simulink model "StampFly_StudentBlocks"  (R2026b)
settings: Solver=VariableStepAuto
undefined symbols (not defined in the file): Bottom, Official
(part 2 of 6)

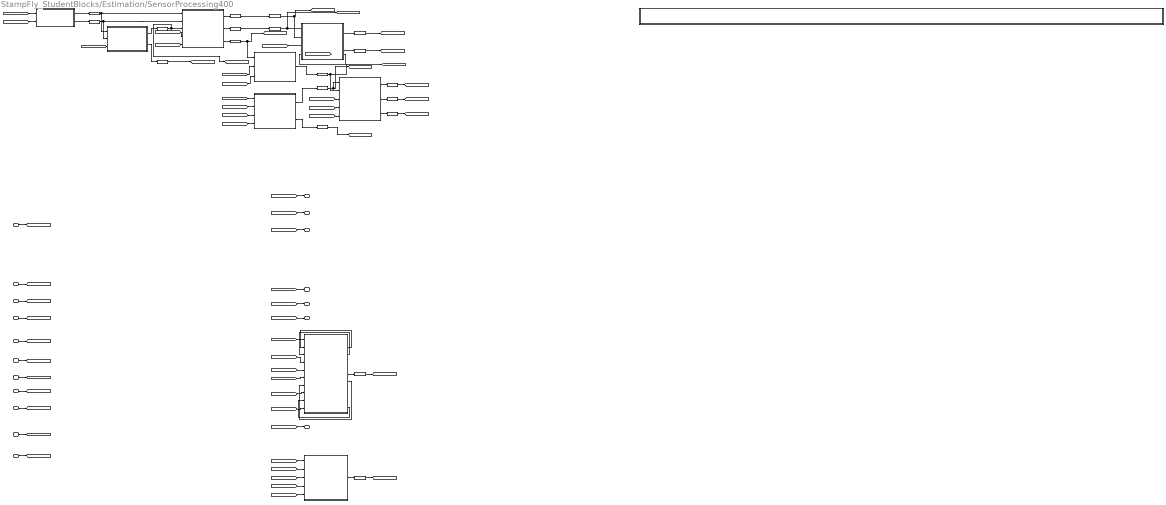
== system StampFly_StudentBlocks/Estimation/SensorProcessing400 ==
  AccelMps2 : Inport
  GyroRps : Inport  Port=2
  ToFmm : Inport  Port=3
  ToFNew : Inport  Port=4
  Voltage : Inport  Port=5
  PreviousMode : Inport  Port=6
  AltFlag : Inport  Port=7
  Dt : Inport  Port=8
  AHRSReset : Inport  Port=9
  ParkingReset : Inport  Port=10
  FlipFlag : Inport  Port=11
  Accel3Size : SignalSpecification  OutDataTypeStr=single  Dimensions=3
  AltitudeKalman : Stateflow chart  Description=高度・鉛直速度・バイアス  TreatAsAtomicUnit=on
      settings: AttributesFormatString=|
      | 高度 Kalman 推定
      | 高度・鉛直速度・バイアス
  Gyro3Size : SignalSpecification  OutDataTypeStr=single  Dimensions=3
  IMUAxisConversion : Stateflow chart  Description=BMI270 → 航空機座標  TreatAsAtomicUnit=on
      settings: AttributesFormatString=|
      | 軸・単位の変換
      | BMI270 → 航空機座標
  IMUBiasCalibration : Stateflow chart  Description=800サンプルでオフセット推定  TreatAsAtomicUnit=on
      settings: AttributesFormatString=|
      | 静止時の校正
      | 800サンプルでオフセット推定
  IMUFiltering : Stateflow chart  Description=校正値を引き一次フィルター  TreatAsAtomicUnit=on
      settings: AttributesFormatString=|
      | IMU フィルター
      | 校正値を引き一次フィルター
  MadgwickAttitude : Stateflow chart  Description=400 Hz / Roll・Pitch・Yaw  TreatAsAtomicUnit=on
      settings: AttributesFormatString=|
      | Madgwick 姿勢推定
      | 400 Hz / Roll・Pitch・Yaw
  ModelExplanation : Subsystem  Description=400 Hz の推定処理：軸変換 → 静止校正 → フィルター → 姿勢推定。下段は ToF と鉛直加速度から高度・上下速度を推定。各ブロックを個別に差し替え可能。
      mask Display: disp('説明\n400 Hz の推定処理：軸変換 → 静止校正 → フィルター → 姿勢推定。下段は ToF と鉛直加速度から高度・上下速度を推定。各ブロックを個別に差し替え可能。')
  SensorDiagnosticPack : Stateflow chart  Description=記録用にまとめる  TreatAsAtomicUnit=on
      settings: AttributesFormatString=|
      | 推定器の診断信号
      | 記録用にまとめる
  SensorFlags : Stateflow chart  Description=距離異常・過加速度・低電圧  TreatAsAtomicUnit=on
      settings: AttributesFormatString=|
      | センサーの状態判定
      | 距離異常・過加速度・低電圧
  ToFHoldOutlierFilter : Stateflow chart  Description=新着距離を判定 / 旧値を保持  TreatAsAtomicUnit=on
      settings: AttributesFormatString=|
      | ToF 保持・外れ値処理
      | 新着距離を判定 / 旧値を保持
  VerticalAcceleration : Stateflow chart  Description=重力成分を除去・フィルター  TreatAsAtomicUnit=on
      settings: AttributesFormatString=|
      | 鉛直加速度
      | 重力成分を除去・フィルター
  spec117_1 : SignalSpecification  OutDataTypeStr=single  Dimensions=3
  spec117_2 : SignalSpecification  OutDataTypeStr=single  Dimensions=3
  spec118_1 : SignalSpecification  OutDataTypeStr=single  Dimensions=4
  spec118_2 : SignalSpecification  OutDataTypeStr=uint16  Dimensions=1
  spec119_1 : SignalSpecification  OutDataTypeStr=single  Dimensions=3
  spec119_2 : SignalSpecification  OutDataTypeStr=single  Dimensions=3
  spec119_3 : SignalSpecification  OutDataTypeStr=single  Dimensions=1
  spec120_1 : SignalSpecification  OutDataTypeStr=single  Dimensions=3
  spec120_2 : SignalSpecification  OutDataTypeStr=single  Dimensions=4
  spec121_1 : SignalSpecification  OutDataTypeStr=single  Dimensions=1
  spec122_1 : SignalSpecification  OutDataTypeStr=single  Dimensions=1
  spec122_2 : SignalSpecification  OutDataTypeStr=int16  Dimensions=1
  spec123_1 : SignalSpecification  OutDataTypeStr=single  Dimensions=1
  spec123_2 : SignalSpecification  OutDataTypeStr=single  Dimensions=1
  spec123_3 : SignalSpecification  OutDataTypeStr=single  Dimensions=1
  spec124_1 : SignalSpecification  OutDataTypeStr=uint8  Dimensions=3
  spec125_1 : SignalSpecification  OutDataTypeStr=single  Dimensions=8
  Attitude3 : Outport  OutDataTypeStr=single  PortDimensions=3
  Rates3 : Outport  Port=2  OutDataTypeStr=single  PortDimensions=3
  Altitude : Outport  Port=3
  Velocity : Outport  Port=4
  Flags3 : Outport  Port=5
  Quaternion4 : Outport  Port=6  OutDataTypeStr=single  PortDimensions=4
  Diagnostics8 : Outport  Port=7
  wires:
  IMUFiltering/2(gf) -> spec119_2/1
  IMUFiltering/1(af) -> spec119_1/1
  IMUBiasCalibration/2(count) -> spec118_2/1
  ToFHoldOutlierFilter/1(alt) -> spec122_1/1
  ToFHoldOutlierFilter/2(raw) -> spec122_2/1
  IMUBiasCalibration/1(offset) -> spec118_1/1
  IMUAxisConversion/2(g) -> spec117_2/1
  IMUAxisConversion/1(a) -> spec117_1/1
  spec117_1/1 -> IMUFiltering/1(a), IMUBiasCalibration/1(a)
  spec117_2/1 -> IMUBiasCalibration/2(g), IMUFiltering/2(g)
  SensorDiagnosticPack/1(diag) -> spec125_1/1
  SensorFlags/1(flags) -> spec124_1/1
  spec125_1/1 -> [diag_S125P1]
  spec124_1/1 -> [flags_S124P1]
  AHRSReset/1 -> [AHRSReset_S83P1]
  FlipFlag/1 -> [FlipFlag_S561P1]
  AltFlag/1 -> [AltFlag_S81P1]
  Voltage/1 -> [Voltage_S79P1]
  ParkingReset/1 -> [ParkingReset_S84P1]
  Dt/1 -> [Dt_S82P1]
  PreviousMode/1 -> [PreviousMode_S80P1]
  ToFNew/1 -> [ToFNew_S78P1]
  ToFmm/1 -> [ToFmm_S77P1]
  GyroRps/1 -> [GyroRps_S76P1]
  AccelMps2/1 -> [AccelMps2_S75P1]
  [Voltage_S79P1] -> SensorFlags/3(voltage)
  [PreviousMode_S80P1] -> SensorFlags/4(mode)
  [AltFlag_S81P1] -> SensorFlags/5(altFlag)
  [Dt_S82P1] -> SensorFlags/8(dt)
  [ParkingReset_S84P1] -> SensorFlags/9(parkingReset)
  [FlipFlag_S561P1] -> SensorFlags/10(flipFlag)
  [af_S119P1] -> SensorFlags/1(accel)
  [gf_S119P2] -> Rates3/1
  [offset_S118P1] -> SensorDiagnosticPack/4(offset)
  [count_S118P2] -> SensorDiagnosticPack/5(count)
  [azd_S119P3] -> SensorFlags/2(azd)
  [a_S120P1] -> Attitude3/1
  [q_S120P2] -> Quaternion4/1
  [az_S121P1] -> SensorDiagnosticPack/1(az)
  [alt_S122P1] -> SensorDiagnosticPack/3(alt)
  [raw_S122P2] -> SensorFlags/7(rawRange)
  [height_S123P1] -> SensorFlags/6(height)
  [height_S123P1] -> Altitude/1
  [velocity_S123P2] -> Velocity/1
  [bias_S123P3] -> SensorDiagnosticPack/2(bias)
  [flags_S124P1] -> Flags3/1
  [diag_S125P1] -> Diagnostics8/1
  spec122_2/1 -> [raw_S122P2]
  spec120_1/1 -> [a_S120P1]
  spec118_2/1 -> [count_S118P2]
  spec118_1/1 -> IMUFiltering/3(offset), [offset_S118P1]
  [AccelMps2_S75P1] -> IMUAxisConversion/1(accelMps2)
  [GyroRps_S76P1] -> IMUAxisConversion/2(gyroRps)
  [ToFmm_S77P1] -> ToFHoldOutlierFilter/1(mm)
  [ToFNew_S78P1] -> ToFHoldOutlierFilter/2(fresh)
  [PreviousMode_S80P1] -> IMUFiltering/4(mode)
  [PreviousMode_S80P1] -> IMUBiasCalibration/3(mode)
  [PreviousMode_S80P1] -> ToFHoldOutlierFilter/3(mode)
  [Dt_S82P1] -> ToFHoldOutlierFilter/4(dt)
  [Dt_S82P1] -> IMUFiltering/5(dt)
  [AHRSReset_S83P1] -> MadgwickAttitude/4(reset)
  [PreviousMode_S80P1] -> MadgwickAttitude/3(mode)
  spec120_2/1 -> [q_S120P2]
  MadgwickAttitude/1(a) -> spec120_1/1
  MadgwickAttitude/2(q) -> spec120_2/1
  VerticalAcceleration/1(az) -> spec121_1/1
  IMUFiltering/3(azd) -> spec119_3/1
  spec119_1/1 -> Accel3Size/1
  spec119_2/1 -> Gyro3Size/1
  spec121_1/1 -> [az_S121P1], AltitudeKalman/2(az)
  spec119_3/1 -> [azd_S119P3], VerticalAcceleration/1(azd)
  Accel3Size/1 -> MadgwickAttitude/2(accel), [af_S119P1]
  Gyro3Size/1 -> MadgwickAttitude/1(rates), [gf_S119P2]
  [PreviousMode_S80P1] -> VerticalAcceleration/2(mode)
  [Dt_S82P1] -> VerticalAcceleration/3(dt)
  [ParkingReset_S84P1] -> AltitudeKalman/5(parkingReset)
  [Dt_S82P1] -> AltitudeKalman/4(dt)
  [PreviousMode_S80P1] -> AltitudeKalman/3(mode)
  spec122_1/1 -> [alt_S122P1], AltitudeKalman/1(alt)
  spec123_1/1 -> [height_S123P1]
  spec123_2/1 -> [velocity_S123P2]
  spec123_3/1 -> [bias_S123P3]
  AltitudeKalman/1(height) -> spec123_1/1
  AltitudeKalman/2(velocity) -> spec123_2/1
  AltitudeKalman/3(bias) -> spec123_3/1

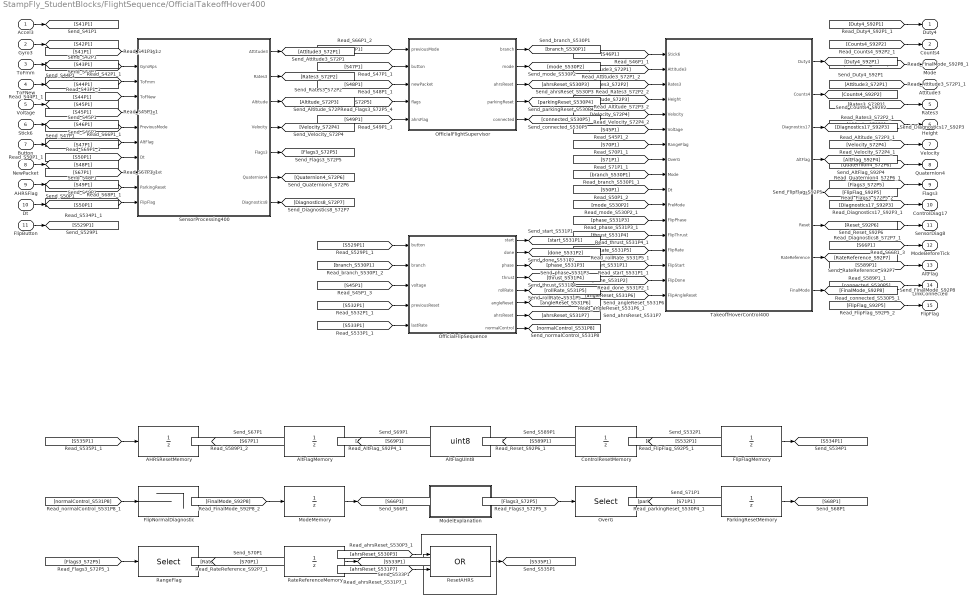
== system StampFly_StudentBlocks/FlightSequence/OfficialTakeoffHover400 ==
  Accel3 : Inport
  Gyro3 : Inport  Port=2
  ToFmm : Inport  Port=3
  ToFNew : Inport  Port=4
  Voltage : Inport  Port=5
  Stick6 : Inport  Port=6
  Button : Inport  Port=7
  NewPacket : Inport  Description=新しいJoyStickパケットをこの周期で受信したか。通信中のフラグとは異なります。  Port=8
  AHRSFlag : Inport  Port=9
  Dt : Inport  Port=10
  FlipButton : Inport  Port=11
  AHRSResetMemory : UnitDelay  InitialCondition=false  SampleTime=Official.Step
  AltFlagMemory : UnitDelay  InitialCondition=uint8(0)  SampleTime=Official.Step
  AltFlagUInt8 : DataTypeConversion  OutDataTypeStr=uint8  SaturateOnIntegerOverflow=off  RndMeth=Floor
  ControlResetMemory : UnitDelay  InitialCondition=false  SampleTime=Official.Step
  FlipFlagMemory : UnitDelay  InitialCondition=uint8(0)  SampleTime=Official.Step
  FlipNormalDiagnostic : Terminator
  ModeMemory : UnitDelay  InitialCondition=uint8(0)  SampleTime=Official.Step
  ModelExplanation : Subsystem  Description=センサー入力 → 推定 → 状態管理 → PID → モーター指令。各ブロックを個別に編集できます。
      mask Display: disp('説明\nセンサー入力 → 推定 → 状態管理 → PID → モーター指令。各ブロックを個別に編集できます。')
  OfficialFlightSupervisor : Stateflow chart  TreatAsAtomicUnit=on
  OfficialFlipSequence : Stateflow chart  TreatAsAtomicUnit=on
  OverG : Selector  InputPortWidth=3  IndexOptions=Index vector (dialog)  Indices=1  OutputSizes=1
  ParkingResetMemory : UnitDelay  InitialCondition=false  SampleTime=Official.Step
  RangeFlag : Selector  InputPortWidth=3  IndexOptions=Index vector (dialog)  Indices=2  OutputSizes=1
  RateReferenceMemory : UnitDelay  InitialCondition=zeros(3,1,'single')  SampleTime=Official.Step
  ResetAHRS : Logic  Operator=OR  AllPortsSameDT=off  OutDataTypeStr=boolean
  SensorProcessing400 : Subsystem  Description=センサー処理：軸変換、800点校正、フィルター、Madgwick、ToF保持/外れ値、高度Kalman、状態フラグを機能別に配置します。
      mask Display: disp('SensorProcessing400\nダブルクリックで内部を編集')
  TakeoffHoverControl400 : Subsystem  Description=飛行制御：目標値→誤差→高度PID/速度PID/姿勢PID/角速度PID→推力制限→ミキサー→8bit化。PIDの内部は標準演算ブロックです。
      mask Display: disp('TakeoffHoverControl400\nダブルクリックで内部を編集')
  Duty4 : Outport
  Counts4 : Outport  Port=2
  Mode : Outport  Port=3
  Attitude3 : Outport  Port=4
  Rates3 : Outport  Port=5
  Height : Outport  Port=6
  Velocity : Outport  Port=7
  Quaternion4 : Outport  Port=8
  Flags3 : Outport  Port=9
  ControlDiag17 : Outport  Port=10
  SensorDiag8 : Outport  Port=11
  ModeBeforeTick : Outport  Port=12
  AltFlag : Outport  Port=13
  LinkConnected : Outport  Port=14
  FlipFlag : Outport  Port=15
  wires:
  TakeoffHoverControl400/8(FinalMode) -> [FinalMode_S92P8]
  TakeoffHoverControl400/7(RateReference) -> [RateReference_S92P7]
  TakeoffHoverControl400/6(Reset) -> [Reset_S92P6]
  TakeoffHoverControl400/5(FlipFlag) -> [FlipFlag_S92P5]
  TakeoffHoverControl400/3(Diagnostics17) -> [Diagnostics17_S92P3]
  TakeoffHoverControl400/2(Counts4) -> [Counts4_S92P2]
  TakeoffHoverControl400/1(Duty4) -> [Duty4_S92P1]
  AltFlagUInt8/1 -> [S589P1]
  ModeMemory/1 -> [S66P1]
  AltFlagMemory/1 -> [S69P1]
  AHRSResetMemory/1 -> [S67P1]
  ParkingResetMemory/1 -> [S68P1]
  SensorProcessing400/5(Flags3) -> [Flags3_S72P5]
  SensorProcessing400/3(Altitude) -> [Altitude_S72P3]
  SensorProcessing400/1(Attitude3) -> [Attitude3_S72P1]
  SensorProcessing400/2(Rates3) -> [Rates3_S72P2]
  SensorProcessing400/4(Velocity) -> [Velocity_S72P4]
  RangeFlag/1 -> [S70P1]
  OverG/1 -> [S71P1]
  SensorProcessing400/6(Quaternion4) -> [Quaternion4_S72P6]
  SensorProcessing400/7(Diagnostics8) -> [Diagnostics8_S72P7]
  ControlResetMemory/1 -> [S532P1]
  RateReferenceMemory/1 -> [S533P1]
  OfficialFlipSequence/3(phase) -> [phase_S531P3]
  OfficialFlipSequence/4(thrust) -> [thrust_S531P4]
  OfficialFlipSequence/5(rollRate) -> [rollRate_S531P5]
  OfficialFlipSequence/1(start) -> [start_S531P1]
  OfficialFlipSequence/2(done) -> [done_S531P2]
  OfficialFlipSequence/6(angleReset) -> [angleReset_S531P6]
  TakeoffHoverControl400/4(AltFlag) -> [AltFlag_S92P4]
  FlipFlagMemory/1 -> [S534P1]
  OfficialFlipSequence/7(ahrsReset) -> [ahrsReset_S531P7]
  ResetAHRS/1 -> [S535P1]
  OfficialFlipSequence/8(normalControl) -> [normalControl_S531P8]
  [S41P1] -> SensorProcessing400/1(AccelMps2)
  [S42P1] -> SensorProcessing400/2(GyroRps)
  [S43P1] -> SensorProcessing400/3(ToFmm)
  [S44P1] -> SensorProcessing400/4(ToFNew)
  [S45P1] -> SensorProcessing400/5(Voltage)
  [S45P1] -> TakeoffHoverControl400/6(Voltage)
  [S45P1] -> OfficialFlipSequence/3(voltage)
  [S46P1] -> TakeoffHoverControl400/1(Stick6)
  [S50P1] -> SensorProcessing400/8(Dt)
  [S50P1] -> TakeoffHoverControl400/10(Dt)
  [S529P1] -> OfficialFlipSequence/1(button)
  [S67P1] -> SensorProcessing400/9(AHRSReset)
  [S69P1] -> SensorProcessing400/7(AltFlag)
  [S589P1] -> AltFlag/1
  [S589P1] -> AltFlagMemory/1
  [S532P1] -> OfficialFlipSequence/4(previousReset)
  [S534P1] -> SensorProcessing400/11(FlipFlag)
  [S66P1] -> SensorProcessing400/6(PreviousMode)
  [S66P1] -> ModeBeforeTick/1
  [branch_S530P1] -> TakeoffHoverControl400/9(Mode)
  [branch_S530P1] -> OfficialFlipSequence/2(branch)
  [mode_S530P2] -> TakeoffHoverControl400/11(PreMode)
  [ahrsReset_S530P3] -> ResetAHRS/1
  [parkingReset_S530P4] -> ParkingResetMemory/1
  [connected_S530P5] -> LinkConnected/1
  [start_S531P1] -> TakeoffHoverControl400/15(FlipStart)
  [done_S531P2] -> TakeoffHoverControl400/16(FlipDone)
  [phase_S531P3] -> TakeoffHoverControl400/12(FlipPhase)
  [thrust_S531P4] -> TakeoffHoverControl400/13(FlipThrust)
  [rollRate_S531P5] -> TakeoffHoverControl400/14(FlipRate)
  [angleReset_S531P6] -> TakeoffHoverControl400/17(FlipAngleReset)
  [ahrsReset_S531P7] -> ResetAHRS/2
  [normalControl_S531P8] -> FlipNormalDiagnostic/1
  [S71P1] -> TakeoffHoverControl400/8(OverG)
  [S68P1] -> SensorProcessing400/10(ParkingReset)
  [S70P1] -> TakeoffHoverControl400/7(RangeFlag)
  [S533P1] -> OfficialFlipSequence/5(lastRate)
  [S535P1] -> AHRSResetMemory/1
  [Attitude3_S72P1] -> Attitude3/1
  [Attitude3_S72P1] -> TakeoffHoverControl400/2(Attitude3)
  [Rates3_S72P2] -> Rates3/1
  [Rates3_S72P2] -> TakeoffHoverControl400/3(Rates3)
  [Altitude_S72P3] -> Height/1
  [Altitude_S72P3] -> TakeoffHoverControl400/4(Height)
  [Velocity_S72P4] -> Velocity/1
  [Velocity_S72P4] -> TakeoffHoverControl400/5(Velocity)
  [Flags3_S72P5] -> RangeFlag/1
  [Flags3_S72P5] -> Flags3/1
  [Flags3_S72P5] -> OverG/1
  [Quaternion4_S72P6] -> Quaternion4/1
  [Diagnostics8_S72P7] -> SensorDiag8/1
  [Duty4_S92P1] -> Duty4/1
  [Counts4_S92P2] -> Counts4/1
  [Diagnostics17_S92P3] -> ControlDiag17/1
  [AltFlag_S92P4] -> AltFlagUInt8/1
  [FlipFlag_S92P5] -> FlipFlagMemory/1
  [FlipFlag_S92P5] -> FlipFlag/1
  [Reset_S92P6] -> ControlResetMemory/1
  [RateReference_S92P7] -> RateReferenceMemory/1
  [FinalMode_S92P8] -> Mode/1
  [FinalMode_S92P8] -> ModeMemory/1
  [Flags3_S72P5] -> OfficialFlightSupervisor/4(flags)
  [S66P1] -> OfficialFlightSupervisor/1(previousMode)
  [S49P1] -> OfficialFlightSupervisor/5(ahrsFlag)
  [S48P1] -> OfficialFlightSupervisor/3(newPacket)
  [S47P1] -> OfficialFlightSupervisor/2(button)
  OfficialFlightSupervisor/3(ahrsReset) -> [ahrsReset_S530P3]
  OfficialFlightSupervisor/5(connected) -> [connected_S530P5]
  OfficialFlightSupervisor/4(parkingReset) -> [parkingReset_S530P4]
  OfficialFlightSupervisor/2(mode) -> [mode_S530P2]
  OfficialFlightSupervisor/1(branch) -> [branch_S530P1]
  Stick6/1 -> [S46P1]
  Accel3/1 -> [S41P1]
  Gyro3/1 -> [S42P1]
  ToFmm/1 -> [S43P1]
  ToFNew/1 -> [S44P1]
  Voltage/1 -> [S45P1]
  Dt/1 -> [S50P1]
  Button/1 -> [S47P1]
  NewPacket/1 -> [S48P1]
  AHRSFlag/1 -> [S49P1]
  FlipButton/1 -> [S529P1]

== system StampFly_StudentBlocks/LoggingAndStatus/DataLogger50 ==
  Accel3 : Inport
  Gyro3 : Inport  Port=2
  IMUFresh : Inport  Port=3
  TimeSec : Inport  Port=4
  BottomMm : Inport  Port=5
  ToFNew : Inport  Port=6
  ToFStatus : Inport  Port=7
  BatteryV : Inport  Port=8
  BatteryValid : Inport  Port=9
  Duty4 : Inport  Port=10
  Mode : Inport  Port=11
  Attitude3 : Inport  Port=12
  Height : Inport  Port=13
  Velocity : Inport  Port=14
  ControlDiag17 : Inport  Port=15
  SensorDiag8 : Inport  Port=16
  ToFInfo4 : Inport  Port=17
  CopiedLoggerSFI8_50 : MATLABSystem  Description=50 Hz SFI8記録：下向きToF距離[m]と状態、ToFValid=(距離>0かつ状態0)。ToFFreshは前回の記録から測定完了数が変化したかで判定。無効時も数値ペイロードと状態を保存し、UIは無効データをNaNで表示。Optical FlowはNaN/無効を保存。高度はSimulinkのKalman出力。  Priority=200  System=official.LoggerPacker50  SimulateUsing=Code generation
      mask Type: official.LoggerPacker50
  ESPNowLogger50 : MATLABSystem  Description=ESP-NOWログ：コピーした受信機のログ形式を使います。送信キュー成功と相手の受信成功は別です。  Priority=221  System=imu.ESPNowIMUTx  Channel=uint8( 3 )  SimulateUsing=Code generation
      mask Type: imu.ESPNowIMUTx
  ModelExplanation : Subsystem  Description=50 Hz SFI8記録：下向きToF距離[m]と状態、ToFValid=(距離>0かつ状態0)。ToFFreshは前回の記録から測定完了数が変化したかで判定。無効時も数値ペイロードと状態を保存し、UIは無効データをNaNで表示。Optical FlowはNaN/無効を保存。高度はSimulinkのKalman出力。
      mask Display: disp('説明\n50 Hz SFI8記録：下向きToF距離[m]と状態、ToFValid=(距離>0かつ状態0)。ToFFreshは前回の記録から測定完了数が変化したかで判定。無効時も数値ペイロードと状態を保存し、UIは無効データをNaNで表示。Optical FlowはNaN/無効を保存。高度はSimulinkのKalman出力。')
  QueuedUSBLogger50 : MATLABSystem  Description=USB送信：待ち時間0でキューへ投入し、別タスクから送信。PCのMATロガーで保存します。  Priority=220  System=official.USBLogger50  SimulateUsing=Code generation
      mask Type: official.USBLogger50
  USBDrops : Outport
  RadioQueued : Outport  Port=2
  LEDMode : Outport  Port=3
  wires:
  Accel3/1 -> CopiedLoggerSFI8_50/1
  Gyro3/1 -> CopiedLoggerSFI8_50/2
  IMUFresh/1 -> CopiedLoggerSFI8_50/3
  TimeSec/1 -> CopiedLoggerSFI8_50/4
  BottomMm/1 -> CopiedLoggerSFI8_50/5
  ToFNew/1 -> CopiedLoggerSFI8_50/6
  ToFStatus/1 -> CopiedLoggerSFI8_50/7
  BatteryV/1 -> CopiedLoggerSFI8_50/8
  BatteryValid/1 -> CopiedLoggerSFI8_50/9
  Duty4/1 -> CopiedLoggerSFI8_50/10
  Mode/1 -> CopiedLoggerSFI8_50/11
  Attitude3/1 -> CopiedLoggerSFI8_50/12
  Height/1 -> CopiedLoggerSFI8_50/13
  Velocity/1 -> CopiedLoggerSFI8_50/14
  ControlDiag17/1 -> CopiedLoggerSFI8_50/15
  SensorDiag8/1 -> CopiedLoggerSFI8_50/16
  ToFInfo4/1 -> CopiedLoggerSFI8_50/17
  CopiedLoggerSFI8_50/1 -> QueuedUSBLogger50/1, ESPNowLogger50/1
  QueuedUSBLogger50/1 -> USBDrops/1
  ESPNowLogger50/1 -> RadioQueued/1
  ESPNowLogger50/2 -> LEDMode/1

== system StampFly_StudentBlocks/LoggingAndStatus/JoyStickTelemetry40 ==
  AltFlag : Inport
  Mode : Inport  Port=2
  FrontMm : Inport  Port=3
  TimeSec : Inport  Port=4
  Dt : Inport  Port=5
  Attitude3 : Inport  Port=6
  Rates3 : Inport  Port=7
  ControlDiag17 : Inport  Port=8
  Accel3 : Inport  Port=9
  BatteryV : Inport  Port=10
  Duty4 : Inport  Port=11
  Height : Inport  Port=12
  SensorDiag8 : Inport  Port=13
  Velocity : Inport  Port=14
  ModelExplanation : Subsystem  Description=JoyStickへ公式テレメトリを40 Hzで返信。高度はSimulinkのKalman出力。前向きToFは無効（0）。
      mask Display: disp('説明\nJoyStickへ公式テレメトリを40 Hzで返信。高度はSimulinkのKalman出力。前向きToFは無効（0）。')
  OfficialHeaderGains20 : Constant  Value=single([.65;.7;.01;.125;.95;.7;.025;.125;3;.8;.01;.125;5;4;.04;.125;5;4;.04;.125])
  OfficialJoyTelemetry40 : MATLABSystem  Description=公式JoyStickへ40 Hzで高度・電圧・姿勢・モード等を返信します。  Priority=240  System=official.RadioTelemetryWrite40  SimulateUsing=Code generation
      mask Type: official.RadioTelemetryWrite40
  OfficialTelemetryValues : Stateflow chart  TreatAsAtomicUnit=on
  Sent : Outport
  wires:
  OfficialJoyTelemetry40/1 -> Sent/1
  Velocity/1 -> OfficialTelemetryValues/11(v)
  SensorDiag8/1 -> OfficialTelemetryValues/10(sd)
  Height/1 -> OfficialTelemetryValues/9(z)
  Duty4/1 -> OfficialTelemetryValues/8(duty)
  BatteryV/1 -> OfficialTelemetryValues/7(voltage)
  Accel3/1 -> OfficialTelemetryValues/6(accel)
  ControlDiag17/1 -> OfficialTelemetryValues/5(cd)
  Rates3/1 -> OfficialTelemetryValues/4(r)
  Attitude3/1 -> OfficialTelemetryValues/3(a)
  Dt/1 -> OfficialTelemetryValues/2(dt)
  TimeSec/1 -> OfficialTelemetryValues/1(t)
  FrontMm/1 -> OfficialJoyTelemetry40/5
  Mode/1 -> OfficialJoyTelemetry40/4
  AltFlag/1 -> OfficialJoyTelemetry40/3
  OfficialHeaderGains20/1 -> OfficialJoyTelemetry40/2
  OfficialTelemetryValues/1(values) -> OfficialJoyTelemetry40/1

== system StampFly_StudentBlocks/LoggingAndStatus/StatusOutputs400 ==
  Stick6 : Inport
  SensorFlags3 : Inport  Port=2
  ModeBeforeTick : Inport  Port=3
  AltFlag : Inport  Port=4
  FlipFlag : Inport  Port=5
  PacketError : Inport  Port=6
  AHRSFlag : Inport  Port=7
  ControlMode : Selector  InputPortWidth=6  IndexOptions=Index vector (dialog)  Indices=5  OutputSizes=1
  LowVoltageCount : Selector  InputPortWidth=3  IndexOptions=Index vector (dialog)  Indices=3  OutputSizes=1
  ModelExplanation : Subsystem  Description=公式のモード・姿勢制御方式・高度制御・Flip・低電圧・通信エラーからLED色とブザー周波数を決定。ハードウェアはキュー送出のみ。
      mask Display: disp('説明\n公式のモード・姿勢制御方式・高度制御・Flip・低電圧・通信エラーからLED色とブザー周波数を決定。ハードウェアはキュー送出のみ。')
  StatusIndicators400 : Stateflow chart  TreatAsAtomicUnit=on
  StatusWrite400 : MATLABSystem  System=official.StatusWrite400  SimulateUsing=Code generation
      mask Type: official.StatusWrite400
  UserButton400 : MATLABSystem  System=official.UserButton400  SimulateUsing=Code generation
      mask Type: official.UserButton400
  wires:
  Stick6/1 -> ControlMode/1
  SensorFlags3/1 -> LowVoltageCount/1
  ModeBeforeTick/1 -> StatusIndicators400/1(mode)
  ControlMode/1 -> StatusIndicators400/2(controlMode)
  AltFlag/1 -> StatusIndicators400/3(altFlag)
  FlipFlag/1 -> StatusIndicators400/4(flipFlag)
  LowVoltageCount/1 -> StatusIndicators400/5(lowVoltage)
  PacketError/1 -> StatusIndicators400/6(rcError)
  AHRSFlag/1 -> StatusIndicators400/7(ahrsFlag)
  UserButton400/1 -> StatusIndicators400/8(button)
  StatusIndicators400/1(color1) -> StatusWrite400/1
  StatusIndicators400/2(color2) -> StatusWrite400/2
  StatusIndicators400/3(tone) -> StatusWrite400/3
  StatusIndicators400/4(restart) -> StatusWrite400/4

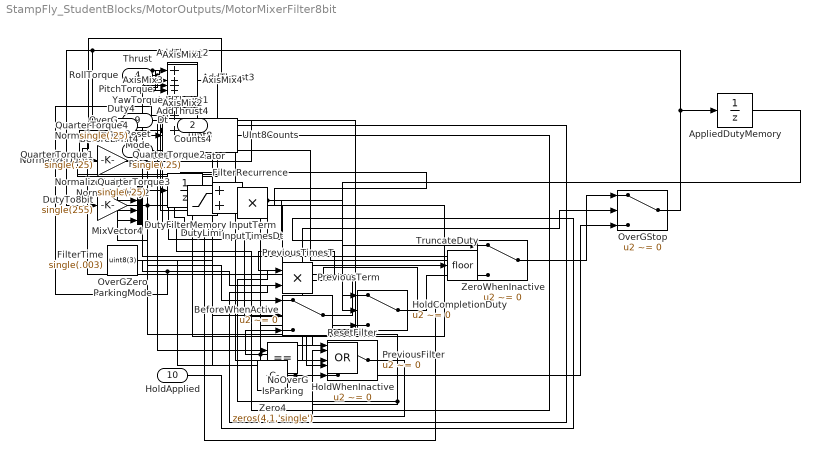
== system StampFly_StudentBlocks/MotorOutputs/MotorMixerFilter8bit ==
  Thrust : Inport
  RollTorque : Inport  Port=2
  PitchTorque : Inport  Port=3
  YawTorque : Inport  Port=4
  Run : Inport  Port=5
  Reset : Inport  Port=6
  OverG : Inport  Port=7
  Mode : Inport  Port=8
  Dt : Inport  Port=9
  HoldApplied : Inport  Port=10
  AddThrust{1..4} (4 alike) : Sum
  AppliedDutyMemory : UnitDelay  InitialCondition=zeros(4,1,'single')  SampleTime=Official.Step
  AxisMix1 : Sum  Inputs=-++
  AxisMix2 : Sum  Inputs=++-
  AxisMix3 : Sum  Inputs=---
  AxisMix4 : Sum  Inputs=+-+
  BeforeWhenActive : Switch  Criteria=u2 ~= 0  SaturateOnIntegerOverflow=off  InputSameDT=off
  DutyFilterMemory : UnitDelay  InitialCondition=zeros(4,1,'single')  SampleTime=Official.Step
  DutyLimit : Saturate  UpperLimit=single(.95)  LowerLimit=single(0)
  DutyTo8bit : Gain  Gain=single(255)
  FilterDenominator : Sum
  FilterRecurrence : Sum
  FilterTime : Constant  Value=single(.003)
  HoldCompletionDuty : Switch  Criteria=u2 ~= 0  SaturateOnIntegerOverflow=off  InputSameDT=off
  HoldWhenInactive : Switch  Criteria=u2 ~= 0  SaturateOnIntegerOverflow=off  InputSameDT=off
  InputTerm : Product  Inputs=*/
  InputTimesDt : Product
  IsParking : RelationalOperator  Operator===  OutDataTypeStr=boolean  RndMeth=Simplest  InputSameDT=off
  MixVector4 : Mux
  NoOverG : RelationalOperator  Operator===  OutDataTypeStr=boolean  RndMeth=Simplest  InputSameDT=off
  NormalizeDuty{1..4} (4 alike) : Gain  Gain=1/3.7  OutDataTypeStr=single
  OverGStop : Switch  Criteria=u2 ~= 0  SaturateOnIntegerOverflow=off  InputSameDT=off
  OverGZero : Constant  Value=uint8(0)
  ParkingMode : Constant  Value=uint8(3)
  PreviousFilter : Switch  Criteria=u2 ~= 0  SaturateOnIntegerOverflow=off  InputSameDT=off
  PreviousTerm : Product  Inputs=*/
  PreviousTimesT : Product
  QuarterTorque{1..4} (4 alike) : Gain  Gain=single(.25)
  ResetFilter : Logic  Operator=OR  AllPortsSameDT=off  OutDataTypeStr=boolean
  TruncateDuty : Rounding
  UInt8Counts : DataTypeConversion  OutDataTypeStr=uint8  SaturateOnIntegerOverflow=off  RndMeth=Floor
  Zero4 : Constant  Value=zeros(4,1,'single')
  ZeroWhenInactive : Switch  Criteria=u2 ~= 0  SaturateOnIntegerOverflow=off  InputSameDT=off
  Duty4 : Outport
  Counts4 : Outport  Port=2
  BeforeLimit4 : Outport  Port=3
  wires:
  RollTorque/1 -> AxisMix2/1, AxisMix3/1, AxisMix1/1, AxisMix4/1
  PitchTorque/1 -> AxisMix1/2, AxisMix2/2, AxisMix3/2, AxisMix4/2
  YawTorque/1 -> AxisMix2/3, AxisMix1/3, AxisMix3/3, AxisMix4/3
  AxisMix1/1 -> QuarterTorque1/1
  Thrust/1 -> AddThrust2/1, AddThrust1/1, AddThrust3/1, AddThrust4/1
  QuarterTorque1/1 -> AddThrust1/2
  AddThrust1/1 -> NormalizeDuty1/1
  AxisMix2/1 -> QuarterTorque2/1
  QuarterTorque2/1 -> AddThrust2/2
  AddThrust2/1 -> NormalizeDuty2/1
  AxisMix3/1 -> QuarterTorque3/1
  QuarterTorque3/1 -> AddThrust3/2
  AddThrust3/1 -> NormalizeDuty3/1
  AxisMix4/1 -> QuarterTorque4/1
  QuarterTorque4/1 -> AddThrust4/2
  AddThrust4/1 -> NormalizeDuty4/1
  Zero4/1 -> OverGStop/3, PreviousFilter/1, BeforeWhenActive/3, HoldCompletionDuty/3
  ResetFilter/1 -> PreviousFilter/2
  DutyFilterMemory/1 -> PreviousFilter/3
  FilterTime/1 -> PreviousTimesT/2, FilterDenominator/1
  PreviousFilter/1 -> PreviousTimesT/1, HoldWhenInactive/3
  PreviousTimesT/1 -> PreviousTerm/1
  FilterDenominator/1 -> PreviousTerm/2, InputTerm/2
  PreviousTerm/1 -> FilterRecurrence/1
  InputTerm/1 -> FilterRecurrence/2
  FilterRecurrence/1 -> DutyLimit/1, HoldWhenInactive/1
  Run/1 -> BeforeWhenActive/2, HoldWhenInactive/2, ZeroWhenInactive/2
  HoldWhenInactive/1 -> DutyFilterMemory/1
  DutyLimit/1 -> ZeroWhenInactive/1
  ZeroWhenInactive/1 -> OverGStop/1
  NoOverG/1 -> OverGStop/2
  OverGStop/1 -> AppliedDutyMemory/1, DutyTo8bit/1, Duty4/1
  DutyTo8bit/1 -> TruncateDuty/1
  TruncateDuty/1 -> UInt8Counts/1
  UInt8Counts/1 -> Counts4/1
  BeforeWhenActive/1 -> BeforeLimit4/1
  NormalizeDuty1/1 -> MixVector4/1
  NormalizeDuty2/1 -> MixVector4/2
  NormalizeDuty3/1 -> MixVector4/3
  NormalizeDuty4/1 -> MixVector4/4
  MixVector4/1 -> InputTimesDt/1, BeforeWhenActive/1
  AppliedDutyMemory/1 -> HoldCompletionDuty/1
  HoldApplied/1 -> HoldCompletionDuty/2
  HoldCompletionDuty/1 -> ZeroWhenInactive/3
  OverGZero/1 -> NoOverG/2
  OverG/1 -> NoOverG/1
  InputTimesDt/1 -> InputTerm/1
  Dt/1 -> FilterDenominator/2, InputTimesDt/2
  Reset/1 -> ResetFilter/2
  IsParking/1 -> ResetFilter/1
  ParkingMode/1 -> IsParking/2
  Mode/1 -> IsParking/1

== system StampFly_StudentBlocks/MotorOutputs/MotorOutputs400 ==
  Counts4 : Inport
  ModelExplanation : Subsystem  Description=入力 Counts4 は FR / FL / RR / RL。LEDCキャリア150 kHz指定・8 bit、指令更新400 Hz。ベンチは定数Enable=falseとAllowMotorOutput=falseで実出力ゼロ。
      mask Display: disp('説明\n入力 Counts4 は FR / FL / RR / RL。LEDCキャリア150 kHz指定・8 bit、指令更新400 Hz。ベンチは定数Enable=falseとAllowMotorOutput=falseで実出力ゼロ。')
  MotorOutputDisabled : Constant  Value=false  SampleTime=Official.Step
  PWM150kHz8bit : MATLABSystem  Description=モーター書き込み：150 kHz指定、8 bit、FR/FL/RR/RL=GPIO42/5/41/10。実機ベンチではAllowMotorOutput=falseかつEnable=false、出力0です。  Priority=100  System=official.MotorPWM400  SampleTime=Official.Step  AllowMotorOutput=false  SimulateUsing=Code generation
      mask Type: official.MotorPWM400
  AppliedCounts4 : Outport
  PWMInfo4 : Outport  Port=2
  wires:
  Counts4/1 -> PWM150kHz8bit/1
  MotorOutputDisabled/1 -> PWM150kHz8bit/2
  PWM150kHz8bit/1 -> AppliedCounts4/1
  PWM150kHz8bit/2 -> PWMInfo4/1

== system StampFly_StudentBlocks/Controllers/TakeoffHoverControl400/AltitudePID ==
  Error : Inport
  Dt : Inport  Port=2
  Enable : Inport  Port=3
  Reset : Inport  Port=4
  PreviousError : Inport  Port=5
  ApplyKp : Product
  DMemory : UnitDelay  InitialCondition=single(0)  SampleTime=Official.Step
  DerivativeDenominator : Sum
  DerivativeErrorProduct : Product
  DerivativeErrorTerm : Product  Inputs=*/
  DerivativePreviousNumerator : Sum  Inputs=+-
  DerivativeUpdate : Sum
  DivideTi : Product  Inputs=*/
  EMemory : UnitDelay  InitialCondition=single(0)  SampleTime=Official.Step
  ErrorDifference : Sum  Inputs=+-
  ErrorPair : Sum
  ErrorPairDt : Product
  Eta : Constant  Value=single(0.125)
  EtaTd : Product
  HalfIntegral : Gain  Gain=single(.5)
  IMemory : UnitDelay  InitialCondition=single(0)  SampleTime=Official.Step
  IntegralLimit : Saturate  UpperLimit=single(30000)  LowerLimit=single(-30000)
  IntegralUpdate : Sum
  Kp : Constant  Value=single(0.379999995)
  PIDTerms : Sum  Inputs=+++
  PreviousDerivativeProduct : Product
  PreviousDerivativeTerm : Product  Inputs=*/
  Select_dnext : Switch  Criteria=u2 ~= 0  SaturateOnIntegerOverflow=off  InputSameDT=off
  Select_dp : Switch  Criteria=u2 ~= 0  SaturateOnIntegerOverflow=off  InputSameDT=off
  Select_enext : Switch  Criteria=u2 ~= 0  SaturateOnIntegerOverflow=off  InputSameDT=off
  Select_ep : Switch  Criteria=u2 ~= 0  SaturateOnIntegerOverflow=off  InputSameDT=off
  Select_inext : Switch  Criteria=u2 ~= 0  SaturateOnIntegerOverflow=off  InputSameDT=off
  Select_ip : Switch  Criteria=u2 ~= 0  SaturateOnIntegerOverflow=off  InputSameDT=off
  Select_output : Switch  Criteria=u2 ~= 0  SaturateOnIntegerOverflow=off  InputSameDT=off
  Select_ynext : Switch  Criteria=u2 ~= 0  SaturateOnIntegerOverflow=off  InputSameDT=off
  Td : Constant  Value=single(0.5)
  Ti : Constant  Value=single(10)
  TwiceEtaTd : Gain  Gain=single(2)
  TwiceTd : Gain  Gain=single(2)
  YMemory : UnitDelay  InitialCondition=single(0)  SampleTime=Official.Step
  Zero : Constant  Value=single(0)
  Output : Outport
  wires:
  Select_output/1 -> Output/1
  Select_ynext/1 -> YMemory/1
  YMemory/1 -> Select_ynext/3, Select_output/3
  ApplyKp/1 -> Select_ynext/1, Select_output/1
  Select_enext/1 -> EMemory/1
  Select_dnext/1 -> DMemory/1
  Select_inext/1 -> IMemory/1
  Enable/1 -> Select_inext/2, Select_dnext/2, Select_enext/2, Select_ynext/2, Select_output/2
  PIDTerms/1 -> ApplyKp/2
  Kp/1 -> ApplyKp/1
  DerivativeUpdate/1 -> PIDTerms/3, Select_dnext/1
  IntegralLimit/1 -> PIDTerms/2, Select_inext/1
  DerivativeErrorTerm/1 -> DerivativeUpdate/2
  PreviousDerivativeTerm/1 -> DerivativeUpdate/1
  DerivativeErrorProduct/1 -> DerivativeErrorTerm/1
  ErrorDifference/1 -> DerivativeErrorProduct/2
  TwiceTd/1 -> DerivativeErrorProduct/1
  DerivativeDenominator/1 -> PreviousDerivativeTerm/2, DerivativeErrorTerm/2
  PreviousDerivativeProduct/1 -> PreviousDerivativeTerm/1
  Select_dp/1 -> PreviousDerivativeProduct/2, Select_dnext/3
  DerivativePreviousNumerator/1 -> PreviousDerivativeProduct/1
  TwiceEtaTd/1 -> DerivativePreviousNumerator/1, DerivativeDenominator/1
  EtaTd/1 -> TwiceEtaTd/1
  Td/1 -> EtaTd/2, TwiceTd/1
  Eta/1 -> EtaTd/1
  IntegralUpdate/1 -> IntegralLimit/1
  DivideTi/1 -> IntegralUpdate/2
  Select_ip/1 -> Select_inext/3, IntegralUpdate/1
  Ti/1 -> DivideTi/2
  HalfIntegral/1 -> DivideTi/1
  ErrorPairDt/1 -> HalfIntegral/1
  ErrorPair/1 -> ErrorPairDt/2
  Dt/1 -> ErrorPairDt/1, DerivativeDenominator/2, DerivativePreviousNumerator/2
  Select_ep/1 -> Select_enext/3, ErrorPair/2, ErrorDifference/2
  Error/1 -> ErrorPair/1, ErrorDifference/1, PIDTerms/1, Select_enext/1
  EMemory/1 -> Select_ep/3
  PreviousError/1 -> Select_ep/1
  DMemory/1 -> Select_dp/3
  IMemory/1 -> Select_ip/3
  Reset/1 -> Select_ip/2, Select_dp/2, Select_ep/2
  Zero/1 -> Select_ip/1, Select_dp/1

== system StampFly_StudentBlocks/Controllers/TakeoffHoverControl400/ModelExplanation ==

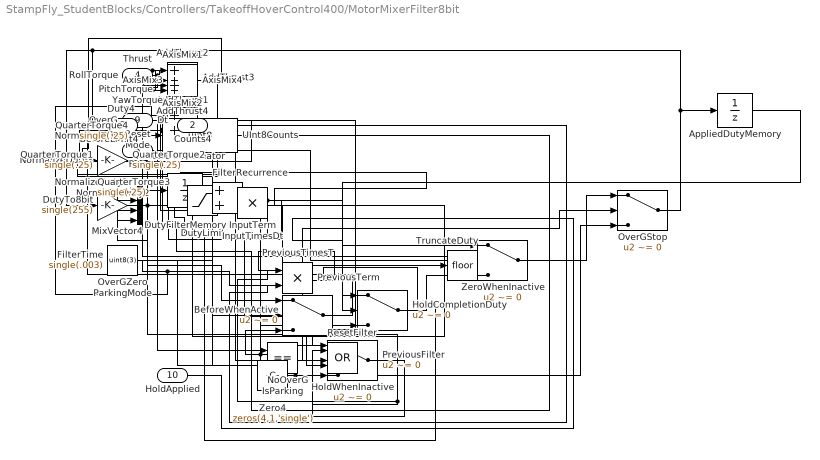
== system StampFly_StudentBlocks/Controllers/TakeoffHoverControl400/MotorMixerFilter8bit ==
  Thrust : Inport
  RollTorque : Inport  Port=2
  PitchTorque : Inport  Port=3
  YawTorque : Inport  Port=4
  Run : Inport  Port=5
  Reset : Inport  Port=6
  OverG : Inport  Port=7
  Mode : Inport  Port=8
  Dt : Inport  Port=9
  HoldApplied : Inport  Port=10
  AddThrust{1..4} (4 alike) : Sum
  AppliedDutyMemory : UnitDelay  InitialCondition=zeros(4,1,'single')  SampleTime=Official.Step
  AxisMix1 : Sum  Inputs=-++
  AxisMix2 : Sum  Inputs=++-
  AxisMix3 : Sum  Inputs=---
  AxisMix4 : Sum  Inputs=+-+
  BeforeWhenActive : Switch  Criteria=u2 ~= 0  SaturateOnIntegerOverflow=off  InputSameDT=off
  DutyFilterMemory : UnitDelay  InitialCondition=zeros(4,1,'single')  SampleTime=Official.Step
  DutyLimit : Saturate  UpperLimit=single(.95)  LowerLimit=single(0)
  DutyTo8bit : Gain  Gain=single(255)
  FilterDenominator : Sum
  FilterRecurrence : Sum
  FilterTime : Constant  Value=single(.003)
  HoldCompletionDuty : Switch  Criteria=u2 ~= 0  SaturateOnIntegerOverflow=off  InputSameDT=off
  HoldWhenInactive : Switch  Criteria=u2 ~= 0  SaturateOnIntegerOverflow=off  InputSameDT=off
  InputTerm : Product  Inputs=*/
  InputTimesDt : Product
  IsParking : RelationalOperator  Operator===  OutDataTypeStr=boolean  RndMeth=Simplest  InputSameDT=off
  MixVector4 : Mux
  NoOverG : RelationalOperator  Operator===  OutDataTypeStr=boolean  RndMeth=Simplest  InputSameDT=off
  NormalizeDuty{1..4} (4 alike) : Gain  Gain=1/3.7  OutDataTypeStr=single
  OverGStop : Switch  Criteria=u2 ~= 0  SaturateOnIntegerOverflow=off  InputSameDT=off
  OverGZero : Constant  Value=uint8(0)
  ParkingMode : Constant  Value=uint8(3)
  PreviousFilter : Switch  Criteria=u2 ~= 0  SaturateOnIntegerOverflow=off  InputSameDT=off
  PreviousTerm : Product  Inputs=*/
  PreviousTimesT : Product
  QuarterTorque{1..4} (4 alike) : Gain  Gain=single(.25)
  ResetFilter : Logic  Operator=OR  AllPortsSameDT=off  OutDataTypeStr=boolean
  TruncateDuty : Rounding
  UInt8Counts : DataTypeConversion  OutDataTypeStr=uint8  SaturateOnIntegerOverflow=off  RndMeth=Floor
  Zero4 : Constant  Value=zeros(4,1,'single')
  ZeroWhenInactive : Switch  Criteria=u2 ~= 0  SaturateOnIntegerOverflow=off  InputSameDT=off
  Duty4 : Outport
  Counts4 : Outport  Port=2
  BeforeLimit4 : Outport  Port=3
  wires:
  RollTorque/1 -> AxisMix2/1, AxisMix3/1, AxisMix1/1, AxisMix4/1
  PitchTorque/1 -> AxisMix1/2, AxisMix2/2, AxisMix3/2, AxisMix4/2
  YawTorque/1 -> AxisMix2/3, AxisMix1/3, AxisMix3/3, AxisMix4/3
  AxisMix1/1 -> QuarterTorque1/1
  Thrust/1 -> AddThrust2/1, AddThrust1/1, AddThrust3/1, AddThrust4/1
  QuarterTorque1/1 -> AddThrust1/2
  AddThrust1/1 -> NormalizeDuty1/1
  AxisMix2/1 -> QuarterTorque2/1
  QuarterTorque2/1 -> AddThrust2/2
  AddThrust2/1 -> NormalizeDuty2/1
  AxisMix3/1 -> QuarterTorque3/1
  QuarterTorque3/1 -> AddThrust3/2
  AddThrust3/1 -> NormalizeDuty3/1
  AxisMix4/1 -> QuarterTorque4/1
  QuarterTorque4/1 -> AddThrust4/2
  AddThrust4/1 -> NormalizeDuty4/1
  Zero4/1 -> OverGStop/3, PreviousFilter/1, BeforeWhenActive/3, HoldCompletionDuty/3
  ResetFilter/1 -> PreviousFilter/2
  DutyFilterMemory/1 -> PreviousFilter/3
  FilterTime/1 -> PreviousTimesT/2, FilterDenominator/1
  PreviousFilter/1 -> PreviousTimesT/1, HoldWhenInactive/3
  PreviousTimesT/1 -> PreviousTerm/1
  FilterDenominator/1 -> PreviousTerm/2, InputTerm/2
  PreviousTerm/1 -> FilterRecurrence/1
  InputTerm/1 -> FilterRecurrence/2
  FilterRecurrence/1 -> DutyLimit/1, HoldWhenInactive/1
  Run/1 -> BeforeWhenActive/2, HoldWhenInactive/2, ZeroWhenInactive/2
  HoldWhenInactive/1 -> DutyFilterMemory/1
  DutyLimit/1 -> ZeroWhenInactive/1
  ZeroWhenInactive/1 -> OverGStop/1
  NoOverG/1 -> OverGStop/2
  OverGStop/1 -> AppliedDutyMemory/1, DutyTo8bit/1, Duty4/1
  DutyTo8bit/1 -> TruncateDuty/1
  TruncateDuty/1 -> UInt8Counts/1
  UInt8Counts/1 -> Counts4/1
  BeforeWhenActive/1 -> BeforeLimit4/1
  NormalizeDuty1/1 -> MixVector4/1
  NormalizeDuty2/1 -> MixVector4/2
  NormalizeDuty3/1 -> MixVector4/3
  NormalizeDuty4/1 -> MixVector4/4
  MixVector4/1 -> InputTimesDt/1, BeforeWhenActive/1
  AppliedDutyMemory/1 -> HoldCompletionDuty/1
  HoldApplied/1 -> HoldCompletionDuty/2
  HoldCompletionDuty/1 -> ZeroWhenInactive/3
  OverGZero/1 -> NoOverG/2
  OverG/1 -> NoOverG/1
  InputTimesDt/1 -> InputTerm/1
  Dt/1 -> FilterDenominator/2, InputTimesDt/2
  Reset/1 -> ResetFilter/2
  IsParking/1 -> ResetFilter/1
  ParkingMode/1 -> IsParking/2
  Mode/1 -> IsParking/1

== system StampFly_StudentBlocks/Controllers/TakeoffHoverControl400/PitchAnglePID ==
  Error : Inport
  Dt : Inport  Port=2
  Enable : Inport  Port=3
  Reset : Inport  Port=4
  PreviousError : Inport  Port=5
  ApplyKp : Product
  DMemory : UnitDelay  InitialCondition=single(0)  SampleTime=Official.Step
  DerivativeDenominator : Sum
  DerivativeErrorProduct : Product
  DerivativeErrorTerm : Product  Inputs=*/
  DerivativePreviousNumerator : Sum  Inputs=+-
  DerivativeUpdate : Sum
  DivideTi : Product  Inputs=*/
  EMemory : UnitDelay  InitialCondition=single(0)  SampleTime=Official.Step
  ErrorDifference : Sum  Inputs=+-
  ErrorPair : Sum
  ErrorPairDt : Product
  Eta : Constant  Value=single(0.125)
  EtaTd : Product
  HalfIntegral : Gain  Gain=single(.5)
  IMemory : UnitDelay  InitialCondition=single(0)  SampleTime=Official.Step
  IntegralLimit : Saturate  UpperLimit=single(30000)  LowerLimit=single(-30000)
  IntegralUpdate : Sum
  Kp : Constant  Value=single(5)
  PIDTerms : Sum  Inputs=+++
  PreviousDerivativeProduct : Product
  PreviousDerivativeTerm : Product  Inputs=*/
  Select_dnext : Switch  Criteria=u2 ~= 0  SaturateOnIntegerOverflow=off  InputSameDT=off
  Select_dp : Switch  Criteria=u2 ~= 0  SaturateOnIntegerOverflow=off  InputSameDT=off
  Select_enext : Switch  Criteria=u2 ~= 0  SaturateOnIntegerOverflow=off  InputSameDT=off
  Select_ep : Switch  Criteria=u2 ~= 0  SaturateOnIntegerOverflow=off  InputSameDT=off
  Select_inext : Switch  Criteria=u2 ~= 0  SaturateOnIntegerOverflow=off  InputSameDT=off
  Select_ip : Switch  Criteria=u2 ~= 0  SaturateOnIntegerOverflow=off  InputSameDT=off
  Select_output : Switch  Criteria=u2 ~= 0  SaturateOnIntegerOverflow=off  InputSameDT=off
  Select_ynext : Switch  Criteria=u2 ~= 0  SaturateOnIntegerOverflow=off  InputSameDT=off
  Td : Constant  Value=single(0.0399999991)
  Ti : Constant  Value=single(4)
  TwiceEtaTd : Gain  Gain=single(2)
  TwiceTd : Gain  Gain=single(2)
  YMemory : UnitDelay  InitialCondition=single(0)  SampleTime=Official.Step
  Zero : Constant  Value=single(0)
  Output : Outport
  wires:
  Enable/1 -> Select_output/2, Select_inext/2, Select_dnext/2, Select_enext/2, Select_ynext/2
  ApplyKp/1 -> Select_ynext/1, Select_output/1
  YMemory/1 -> Select_ynext/3, Select_output/3
  Select_ynext/1 -> YMemory/1
  Select_output/1 -> Output/1
  Select_enext/1 -> EMemory/1
  Select_dnext/1 -> DMemory/1
  Select_inext/1 -> IMemory/1
  PIDTerms/1 -> ApplyKp/2
  Kp/1 -> ApplyKp/1
  DerivativeUpdate/1 -> PIDTerms/3, Select_dnext/1
  IntegralLimit/1 -> PIDTerms/2, Select_inext/1
  DerivativeErrorTerm/1 -> DerivativeUpdate/2
  PreviousDerivativeTerm/1 -> DerivativeUpdate/1
  DerivativeErrorProduct/1 -> DerivativeErrorTerm/1
  ErrorDifference/1 -> DerivativeErrorProduct/2
  TwiceTd/1 -> DerivativeErrorProduct/1
  DerivativeDenominator/1 -> PreviousDerivativeTerm/2, DerivativeErrorTerm/2
  PreviousDerivativeProduct/1 -> PreviousDerivativeTerm/1
  Select_dp/1 -> PreviousDerivativeProduct/2, Select_dnext/3
  DerivativePreviousNumerator/1 -> PreviousDerivativeProduct/1
  TwiceEtaTd/1 -> DerivativePreviousNumerator/1, DerivativeDenominator/1
  EtaTd/1 -> TwiceEtaTd/1
  Td/1 -> EtaTd/2, TwiceTd/1
  Eta/1 -> EtaTd/1
  IntegralUpdate/1 -> IntegralLimit/1
  DivideTi/1 -> IntegralUpdate/2
  Select_ip/1 -> Select_inext/3, IntegralUpdate/1
  Ti/1 -> DivideTi/2
  HalfIntegral/1 -> DivideTi/1
  ErrorPairDt/1 -> HalfIntegral/1
  ErrorPair/1 -> ErrorPairDt/2
  Dt/1 -> ErrorPairDt/1, DerivativeDenominator/2, DerivativePreviousNumerator/2
  Select_ep/1 -> Select_enext/3, ErrorPair/2, ErrorDifference/2
  Error/1 -> ErrorPair/1, ErrorDifference/1, PIDTerms/1, Select_enext/1
  EMemory/1 -> Select_ep/3
  PreviousError/1 -> Select_ep/1
  DMemory/1 -> Select_dp/3
  IMemory/1 -> Select_ip/3
  Reset/1 -> Select_ip/2, Select_dp/2, Select_ep/2
  Zero/1 -> Select_ip/1, Select_dp/1

== system StampFly_StudentBlocks/Controllers/TakeoffHoverControl400/PitchRatePID ==
  Error : Inport
  Dt : Inport  Port=2
  Enable : Inport  Port=3
  Reset : Inport  Port=4
  PreviousError : Inport  Port=5
  ApplyKp : Product
  DMemory : UnitDelay  InitialCondition=single(0)  SampleTime=Official.Step
  DerivativeDenominator : Sum
  DerivativeErrorProduct : Product
  DerivativeErrorTerm : Product  Inputs=*/
  DerivativePreviousNumerator : Sum  Inputs=+-
  DerivativeUpdate : Sum
  DivideTi : Product  Inputs=*/
  EMemory : UnitDelay  InitialCondition=single(0)  SampleTime=Official.Step
  ErrorDifference : Sum  Inputs=+-
  ErrorPair : Sum
  ErrorPairDt : Product
  Eta : Constant  Value=single(0.125)
  EtaTd : Product
  HalfIntegral : Gain  Gain=single(.5)
  IMemory : UnitDelay  InitialCondition=single(0)  SampleTime=Official.Step
  IntegralLimit : Saturate  UpperLimit=single(30000)  LowerLimit=single(-30000)
  IntegralUpdate : Sum
  Kp : Constant  Value=single(0.949999988)
  PIDTerms : Sum  Inputs=+++
  PreviousDerivativeProduct : Product
  PreviousDerivativeTerm : Product  Inputs=*/
  Select_dnext : Switch  Criteria=u2 ~= 0  SaturateOnIntegerOverflow=off  InputSameDT=off
  Select_dp : Switch  Criteria=u2 ~= 0  SaturateOnIntegerOverflow=off  InputSameDT=off
  Select_enext : Switch  Criteria=u2 ~= 0  SaturateOnIntegerOverflow=off  InputSameDT=off
  Select_ep : Switch  Criteria=u2 ~= 0  SaturateOnIntegerOverflow=off  InputSameDT=off
  Select_inext : Switch  Criteria=u2 ~= 0  SaturateOnIntegerOverflow=off  InputSameDT=off
  Select_ip : Switch  Criteria=u2 ~= 0  SaturateOnIntegerOverflow=off  InputSameDT=off
  Select_output : Switch  Criteria=u2 ~= 0  SaturateOnIntegerOverflow=off  InputSameDT=off
  Select_ynext : Switch  Criteria=u2 ~= 0  SaturateOnIntegerOverflow=off  InputSameDT=off
  Td : Constant  Value=single(0.0250000004)
  Ti : Constant  Value=single(0.699999988)
  TwiceEtaTd : Gain  Gain=single(2)
  TwiceTd : Gain  Gain=single(2)
  YMemory : UnitDelay  InitialCondition=single(0)  SampleTime=Official.Step
  Zero : Constant  Value=single(0)
  Output : Outport
  wires:
  Enable/1 -> Select_output/2, Select_inext/2, Select_dnext/2, Select_enext/2, Select_ynext/2
  ApplyKp/1 -> Select_ynext/1, Select_output/1
  YMemory/1 -> Select_ynext/3, Select_output/3
  Select_ynext/1 -> YMemory/1
  Select_output/1 -> Output/1
  Select_enext/1 -> EMemory/1
  Select_dnext/1 -> DMemory/1
  Select_inext/1 -> IMemory/1
  PIDTerms/1 -> ApplyKp/2
  Kp/1 -> ApplyKp/1
  DerivativeUpdate/1 -> PIDTerms/3, Select_dnext/1
  IntegralLimit/1 -> PIDTerms/2, Select_inext/1
  DerivativeErrorTerm/1 -> DerivativeUpdate/2
  PreviousDerivativeTerm/1 -> DerivativeUpdate/1
  DerivativeErrorProduct/1 -> DerivativeErrorTerm/1
  ErrorDifference/1 -> DerivativeErrorProduct/2
  TwiceTd/1 -> DerivativeErrorProduct/1
  DerivativeDenominator/1 -> PreviousDerivativeTerm/2, DerivativeErrorTerm/2
  PreviousDerivativeProduct/1 -> PreviousDerivativeTerm/1
  Select_dp/1 -> PreviousDerivativeProduct/2, Select_dnext/3
  DerivativePreviousNumerator/1 -> PreviousDerivativeProduct/1
  TwiceEtaTd/1 -> DerivativePreviousNumerator/1, DerivativeDenominator/1
  EtaTd/1 -> TwiceEtaTd/1
  Td/1 -> EtaTd/2, TwiceTd/1
  Eta/1 -> EtaTd/1
  IntegralUpdate/1 -> IntegralLimit/1
  DivideTi/1 -> IntegralUpdate/2
  Select_ip/1 -> Select_inext/3, IntegralUpdate/1
  Ti/1 -> DivideTi/2
  HalfIntegral/1 -> DivideTi/1
  ErrorPairDt/1 -> HalfIntegral/1
  ErrorPair/1 -> ErrorPairDt/2
  Dt/1 -> ErrorPairDt/1, DerivativeDenominator/2, DerivativePreviousNumerator/2
  Select_ep/1 -> Select_enext/3, ErrorPair/2, ErrorDifference/2
  Error/1 -> ErrorPair/1, ErrorDifference/1, PIDTerms/1, Select_enext/1
  EMemory/1 -> Select_ep/3
  PreviousError/1 -> Select_ep/1
  DMemory/1 -> Select_dp/3
  IMemory/1 -> Select_ip/3
  Reset/1 -> Select_ip/2, Select_dp/2, Select_ep/2
  Zero/1 -> Select_ip/1, Select_dp/1

== system StampFly_StudentBlocks/Controllers/TakeoffHoverControl400/RollAnglePID ==
  Error : Inport
  Dt : Inport  Port=2
  Enable : Inport  Port=3
  Reset : Inport  Port=4
  PreviousError : Inport  Port=5
  ApplyKp : Product
  DMemory : UnitDelay  InitialCondition=single(0)  SampleTime=Official.Step
  DerivativeDenominator : Sum
  DerivativeErrorProduct : Product
  DerivativeErrorTerm : Product  Inputs=*/
  DerivativePreviousNumerator : Sum  Inputs=+-
  DerivativeUpdate : Sum
  DivideTi : Product  Inputs=*/
  EMemory : UnitDelay  InitialCondition=single(0)  SampleTime=Official.Step
  ErrorDifference : Sum  Inputs=+-
  ErrorPair : Sum
  ErrorPairDt : Product
  Eta : Constant  Value=single(0.125)
  EtaTd : Product
  HalfIntegral : Gain  Gain=single(.5)
  IMemory : UnitDelay  InitialCondition=single(0)  SampleTime=Official.Step
  IntegralLimit : Saturate  UpperLimit=single(30000)  LowerLimit=single(-30000)
  IntegralUpdate : Sum
  Kp : Constant  Value=single(5)
  PIDTerms : Sum  Inputs=+++
  PreviousDerivativeProduct : Product
  PreviousDerivativeTerm : Product  Inputs=*/
  Select_dnext : Switch  Criteria=u2 ~= 0  SaturateOnIntegerOverflow=off  InputSameDT=off
  Select_dp : Switch  Criteria=u2 ~= 0  SaturateOnIntegerOverflow=off  InputSameDT=off
  Select_enext : Switch  Criteria=u2 ~= 0  SaturateOnIntegerOverflow=off  InputSameDT=off
  Select_ep : Switch  Criteria=u2 ~= 0  SaturateOnIntegerOverflow=off  InputSameDT=off
  Select_inext : Switch  Criteria=u2 ~= 0  SaturateOnIntegerOverflow=off  InputSameDT=off
  Select_ip : Switch  Criteria=u2 ~= 0  SaturateOnIntegerOverflow=off  InputSameDT=off
  Select_output : Switch  Criteria=u2 ~= 0  SaturateOnIntegerOverflow=off  InputSameDT=off
  Select_ynext : Switch  Criteria=u2 ~= 0  SaturateOnIntegerOverflow=off  InputSameDT=off
  Td : Constant  Value=single(0.0399999991)
  Ti : Constant  Value=single(4)
  TwiceEtaTd : Gain  Gain=single(2)
  TwiceTd : Gain  Gain=single(2)
  YMemory : UnitDelay  InitialCondition=single(0)  SampleTime=Official.Step
  Zero : Constant  Value=single(0)
  Output : Outport
  wires:
  Enable/1 -> Select_output/2, Select_inext/2, Select_dnext/2, Select_enext/2, Select_ynext/2
  ApplyKp/1 -> Select_ynext/1, Select_output/1
  YMemory/1 -> Select_ynext/3, Select_output/3
  Select_ynext/1 -> YMemory/1
  Select_output/1 -> Output/1
  Select_enext/1 -> EMemory/1
  Select_dnext/1 -> DMemory/1
  Select_inext/1 -> IMemory/1
  PIDTerms/1 -> ApplyKp/2
  Kp/1 -> ApplyKp/1
  DerivativeUpdate/1 -> PIDTerms/3, Select_dnext/1
  IntegralLimit/1 -> PIDTerms/2, Select_inext/1
  DerivativeErrorTerm/1 -> DerivativeUpdate/2
  PreviousDerivativeTerm/1 -> DerivativeUpdate/1
  DerivativeErrorProduct/1 -> DerivativeErrorTerm/1
  ErrorDifference/1 -> DerivativeErrorProduct/2
  TwiceTd/1 -> DerivativeErrorProduct/1
  DerivativeDenominator/1 -> PreviousDerivativeTerm/2, DerivativeErrorTerm/2
  PreviousDerivativeProduct/1 -> PreviousDerivativeTerm/1
  Select_dp/1 -> PreviousDerivativeProduct/2, Select_dnext/3
  DerivativePreviousNumerator/1 -> PreviousDerivativeProduct/1
  TwiceEtaTd/1 -> DerivativePreviousNumerator/1, DerivativeDenominator/1
  EtaTd/1 -> TwiceEtaTd/1
  Td/1 -> EtaTd/2, TwiceTd/1
  Eta/1 -> EtaTd/1
  IntegralUpdate/1 -> IntegralLimit/1
  DivideTi/1 -> IntegralUpdate/2
  Select_ip/1 -> Select_inext/3, IntegralUpdate/1
  Ti/1 -> DivideTi/2
  HalfIntegral/1 -> DivideTi/1
  ErrorPairDt/1 -> HalfIntegral/1
  ErrorPair/1 -> ErrorPairDt/2
  Dt/1 -> ErrorPairDt/1, DerivativeDenominator/2, DerivativePreviousNumerator/2
  Select_ep/1 -> Select_enext/3, ErrorPair/2, ErrorDifference/2
  Error/1 -> ErrorPair/1, ErrorDifference/1, PIDTerms/1, Select_enext/1
  EMemory/1 -> Select_ep/3
  PreviousError/1 -> Select_ep/1
  DMemory/1 -> Select_dp/3
  IMemory/1 -> Select_ip/3
  Reset/1 -> Select_ip/2, Select_dp/2, Select_ep/2
  Zero/1 -> Select_ip/1, Select_dp/1
